simulink model "ParId_V_m_model"  (R2026b)
settings: Solver=VariableStepAuto
undefined symbols (not defined in the file): p_a, p_m, params
settings Model: Creator=User  LastModifiedBy=Mauro

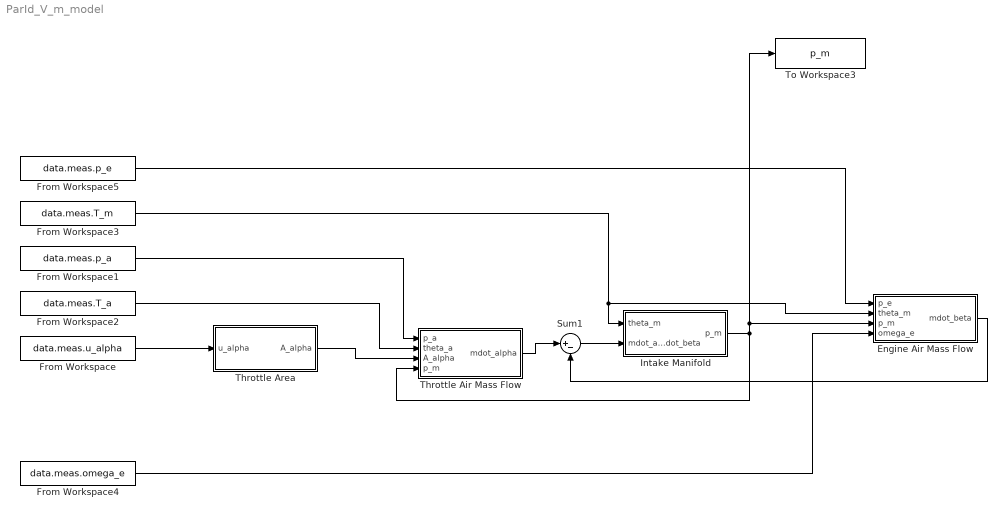
== system ParId_V_m_model ==
  Engine Air Mass Flow : Subsystem
  From Workspace : FromWorkspace  VariableName=data.meas.u_alpha
  From Workspace1 : FromWorkspace  VariableName=data.meas.p_a
  From Workspace2 : FromWorkspace  VariableName=data.meas.T_a
  From Workspace3 : FromWorkspace  VariableName=data.meas.T_m
  From Workspace4 : FromWorkspace  VariableName=data.meas.omega_e
  From Workspace5 : FromWorkspace  VariableName=data.meas.p_e
  Intake Manifold : Subsystem
  Sum1 : Sum  Inputs=|+-
  Throttle Air Mass Flow : Subsystem
  Throttle Area : Subsystem
  To Workspace3 : ToWorkspace  VariableName=p_m  SaveFormat=Timeseries  SampleTime=-1
  wires:
  From Workspace5/1 -> Engine Air Mass Flow/1(p_e)
  Throttle Area/1(A_alpha) -> Throttle Air Mass Flow/3(A_alpha)
  From Workspace1/1 -> Throttle Air Mass Flow/1(p_a)
  Sum1/1 -> Intake Manifold/2(mdot_alpha-mdot_beta)
  From Workspace3/1 -> Engine Air Mass Flow/2(theta_m), Intake Manifold/1(theta_m)
  Throttle Air Mass Flow/1(mdot_alpha) -> Sum1/1
  Intake Manifold/1(p_m) -> To Workspace3/1, Engine Air Mass Flow/3(p_m), Throttle Air Mass Flow/4(p_m)
  Engine Air Mass Flow/1(mdot_beta) -> Sum1/2
  From Workspace4/1 -> Engine Air Mass Flow/4(omega_e)
  From Workspace/1 -> Throttle Area/1(u_alpha)
  From Workspace2/1 -> Throttle Air Mass Flow/2(theta_a)

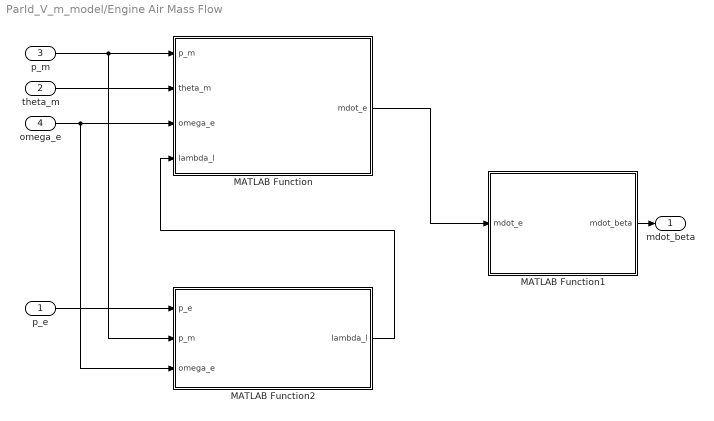
== system ParId_V_m_model/Engine Air Mass Flow ==
  p_e : Inport
  theta_m : Inport  Port=2
  p_m : Inport  Port=3
  omega_e : Inport  Port=4
  MATLAB Function : MATLAB Function  TreatAsAtomicUnit=on
  MATLAB Function1 : MATLAB Function  TreatAsAtomicUnit=on
  MATLAB Function2 : MATLAB Function  TreatAsAtomicUnit=on
  mdot_beta : Outport
  wires:
  MATLAB Function2/1(lambda_l) -> MATLAB Function/4(lambda_l)
  MATLAB Function1/1(mdot_beta) -> mdot_beta/1
  theta_m/1 -> MATLAB Function/2(theta_m)
  p_e/1 -> MATLAB Function2/1(p_e)
  p_m/1 -> MATLAB Function2/2(p_m), MATLAB Function/1(p_m)
  MATLAB Function/1(mdot_e) -> MATLAB Function1/1(mdot_e)
  omega_e/1 -> MATLAB Function/3(omega_e), MATLAB Function2/3(omega_e)

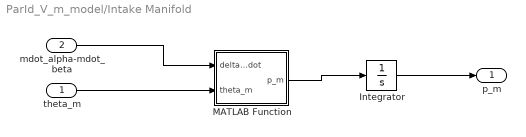
== system ParId_V_m_model/Intake Manifold ==
  theta_m : Inport
  mdot_alpha-mdot_beta : Inport  Port=2
  Integrator : Integrator  InitialCondition=params.p_m0
  MATLAB Function : MATLAB Function  TreatAsAtomicUnit=on
  p_m : Outport
  wires:
  Integrator/1 -> p_m/1
  mdot_alpha-mdot_beta/1 -> MATLAB Function/1(delta_mdot)
  theta_m/1 -> MATLAB Function/2(theta_m)
  MATLAB Function/1(p_m) -> Integrator/1

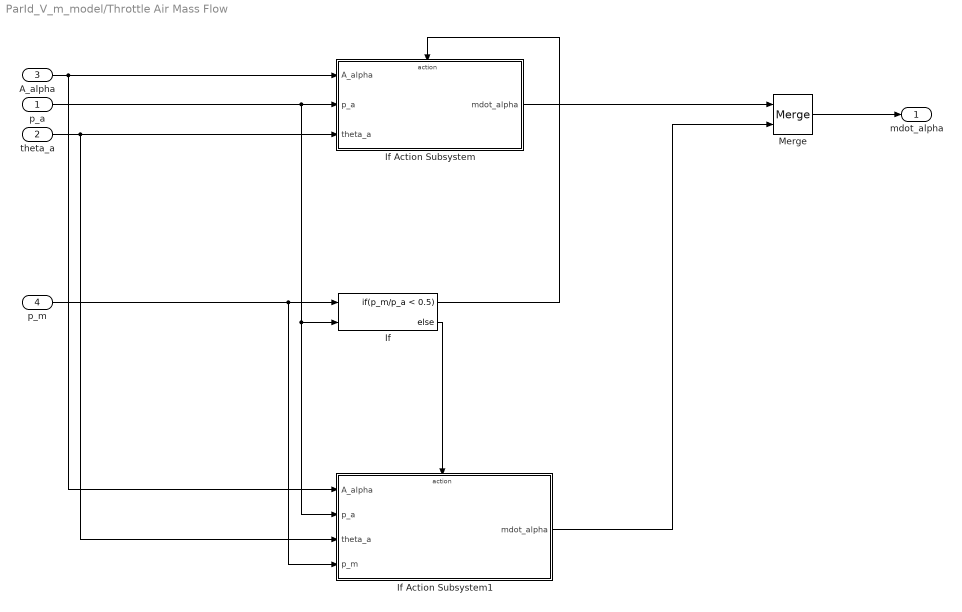
== system ParId_V_m_model/Throttle Air Mass Flow ==
  p_a : Inport
  theta_a : Inport  Port=2
  A_alpha : Inport  Port=3
  p_m : Inport  Port=4
  If : If  NumInputs=2  IfExpression=p_m/p_a < 0.5  InportLabels=p_m,p_a
  If Action Subsystem : Subsystem  TreatAsAtomicUnit=on
  If Action Subsystem1 : Subsystem  TreatAsAtomicUnit=on
  Merge : Merge
  mdot_alpha : Outport
  wires:
  theta_a/1 -> If Action Subsystem/3(theta_a), If Action Subsystem1/3(theta_a)
  Merge/1 -> mdot_alpha/1
  If Action Subsystem/1(mdot_alpha) -> Merge/1
  p_a/1 -> If/2, If Action Subsystem1/2(p_a), If Action Subsystem/2(p_a)
  A_alpha/1 -> If Action Subsystem/1(A_alpha), If Action Subsystem1/1(A_alpha)
  If/2 -> If Action Subsystem1/Action
  If Action Subsystem1/1(mdot_alpha) -> Merge/2
  p_m/1 -> If/1, If Action Subsystem1/4(p_m)
  If/1 -> If Action Subsystem/Action

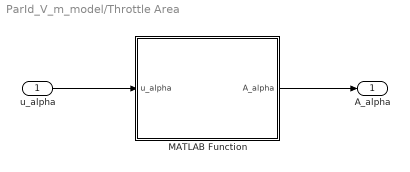
== system ParId_V_m_model/Throttle Area ==
  u_alpha : Inport
  MATLAB Function : MATLAB Function  TreatAsAtomicUnit=on
  A_alpha : Outport
  wires:
  u_alpha/1 -> MATLAB Function/1(u_alpha)
  MATLAB Function/1(A_alpha) -> A_alpha/1

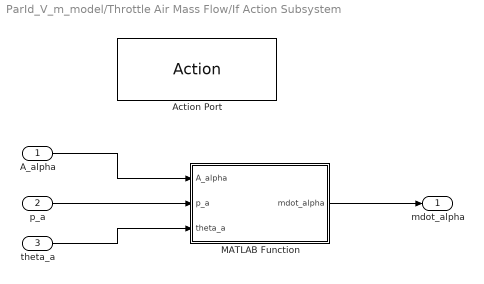
== system ParId_V_m_model/Throttle Air Mass Flow/If Action Subsystem ==
  A_alpha : Inport
  p_a : Inport  Port=2
  theta_a : Inport  Port=3
  Action Port : ActionPort  ActionPortLabel=if(p_m/p_a < 0.5)
  MATLAB Function : MATLAB Function  TreatAsAtomicUnit=on
  mdot_alpha : Outport
  wires:
  A_alpha/1 -> MATLAB Function/1(A_alpha)
  p_a/1 -> MATLAB Function/2(p_a)
  theta_a/1 -> MATLAB Function/3(theta_a)
  MATLAB Function/1(mdot_alpha) -> mdot_alpha/1

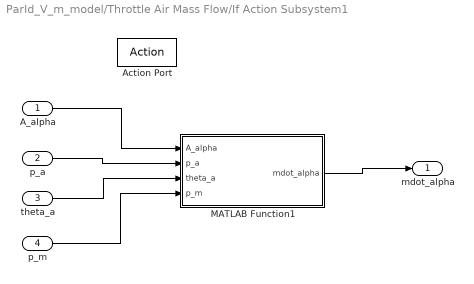
== system ParId_V_m_model/Throttle Air Mass Flow/If Action Subsystem1 ==
  A_alpha : Inport
  p_a : Inport  Port=2
  theta_a : Inport  Port=3
  p_m : Inport  Port=4
  Action Port : ActionPort  ActionPortLabel=else
  MATLAB Function1 : MATLAB Function  TreatAsAtomicUnit=on
  mdot_alpha : Outport
  wires:
  A_alpha/1 -> MATLAB Function1/1(A_alpha)
  p_a/1 -> MATLAB Function1/2(p_a)
  theta_a/1 -> MATLAB Function1/3(theta_a)
  p_m/1 -> MATLAB Function1/4(p_m)
  MATLAB Function1/1(mdot_alpha) -> mdot_alpha/1

== matlab function ParId_V_m_model/Intake Manifold/MATLAB Function ==
  data: delta_mdot input; theta_m input; p_m output; params parameter
function p_m = fcn(delta_mdot, theta_m, params)

p_m = delta_mdot * theta_m * params.R / params.Vm;

== matlab function ParId_V_m_model/Throttle Air Mass Flow/If Action Subsystem/MATLAB Function ==
  data: A_alpha input; mdot_alpha output; p_a input; theta_a input; params parameter
function mdot_alpha = fcn(A_alpha,p_a,theta_a, params)

mdot_alpha = A_alpha * p_a/sqrt(params.R*theta_a) * 1/sqrt(2);

== matlab function ParId_V_m_model/Throttle Air Mass Flow/If Action Subsystem1/MATLAB Function1 ==
  data: A_alpha input; mdot_alpha output; p_a input; theta_a input; p_m input; params parameter
function mdot_alpha = fcn(A_alpha, p_a, theta_a, p_m, params)

% if p_m/p_a >=1
%     mdot_alpha = 1;
%     fprintf('\nratio greater 1')
% else
%     mdot_alpha = A_alpha * p_a / sqrt(params.R * theta_a) * sqrt((2*p_m/p_a)*(1-p_m/p_a));
% end

mdot_alpha = A_alpha * p_a / sqrt(params.R * theta_a) * sqrt((2*p_m/p_a)*(1-p_m/p_a));

== matlab function ParId_V_m_model/Throttle Area/MATLAB Function ==
  data: u_alpha input; A_alpha output; params parameter
function A_alpha = fcn(u_alpha, params)

A_alpha = params.alpha_0 + params.alpha_1*u_alpha;

== matlab function ParId_V_m_model/Engine Air Mass Flow/MATLAB Function ==
  data: mdot_e output; p_m input; theta_m input; omega_e input; lambda_l input; params parameter
function mdot_e = FreshMixtureMassFlow(p_m, theta_m, omega_e, lambda_l, params)

% Fresh mixture that enters the cylinder

mdot_e = 1/2 ... 
         * p_m/(params.R*theta_m) ...
         * lambda_l ...
         * params.V_d ... 
         * omega_e/(2*pi);

end

== matlab function ParId_V_m_model/Engine Air Mass Flow/MATLAB Function1 ==
  data: mdot_beta output; mdot_e input; params parameter
function mdot_beta = MixtureToAirMassFlow(mdot_e, params)

% Air mass flow out of the intake manifold

mdot_beta = mdot_e / (1 + (1 / (params.lambda * params.sigma_0)));

end

== matlab function ParId_V_m_model/Engine Air Mass Flow/MATLAB Function2 ==
  data: p_e input; lambda_l output; p_m input; omega_e input; params parameter
function lambda_l = VolumetricEfficiency(p_e, p_m, omega_e, params)

% Volumetric efficiency

lambda_lp = (params.V_c + params.V_d)/params.V_d ...
            - params.V_c/params.V_d ...
            * (p_e/p_m)^(1/params.kappa);

lambda_lomega = params.gamma_0 + params.gamma_1 * omega_e;

lambda_l = lambda_lp * lambda_lomega;

end
